simulink model "BMS_Dashboard"  (R2025b)
settings: Solver=FixedStepDiscrete  StartTime=0.0  StopTime=300  FixedStep=Ts  RelTol=1e-3
InitFcn:
  | init_BMS
undefined symbols (not defined in the file): Ts
libraries: BMS_Library x1
settings Model: Creator=Khadija  LastModifiedBy=Khadija

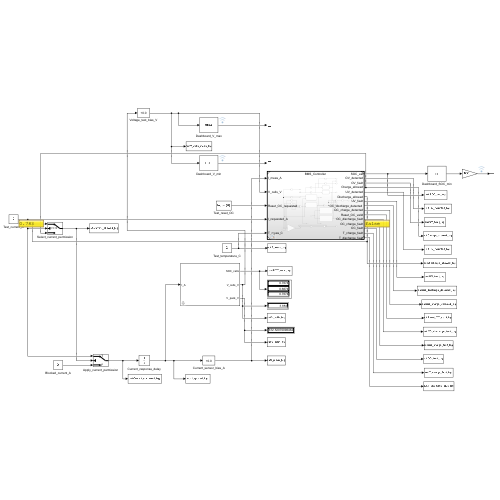
[thumbnail: Simulink's stored preview of the top-level diagram]
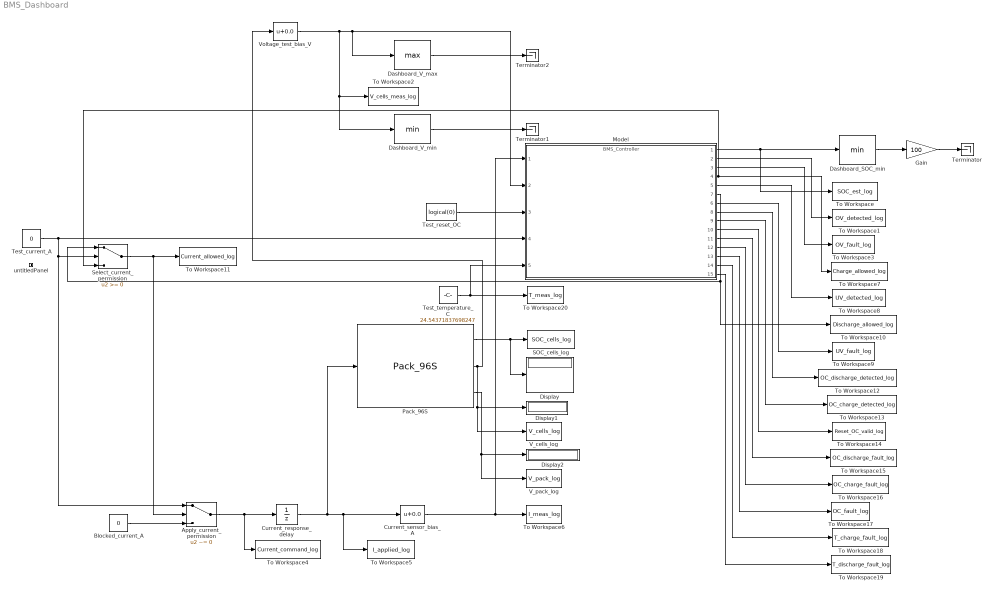
== system BMS_Dashboard ==
  Apply_current_permission : Switch  Criteria=u2 ~= 0  SaturateOnIntegerOverflow=off  InputSameDT=off
  Blocked_current_A : Constant  Value=0  SampleTime=Ts
  Current_response_delay : UnitDelay  SampleTime=Ts  HasFrameUpgradeWarning=on
  Current_sensor_bias_A : Bias  Bias=0.0  SaturateOnIntegerOverflow=off
  Dashboard_SOC_min : MinMax
  Dashboard_V_max : MinMax  Function=max
  Dashboard_V_min : MinMax
  Display : Display
  Display1 : Display
  Display2 : Display
  Gain : Gain  Gain=100
  Model : ModelReference  ModelNameDialog=BMS_Controller  SimulationMode=Normal  ModelReferenceVersion=1.40
      settings: PortSchema="{\"entries\":[{\"content\":{\"sides\":[{\"content\":{\"connectorIds\":[\"In1\",\"In2\",\"In3\",\"In4\",\"In5\"]},\"type\":\"ConnectorPlacement.EquallySpacedRectSide\",\"uuid\":\"1e26f145-0f3d-496d-921d-7ad329268fcb\"},{\"content\":{\"connectorIds\":[\"Out1\",\"Out2\",\"Out3\",\"Out4\",\"Out5\",\"Out7\",\"Out6\",\"Out8\",\"Out9\",\"Out10\",\"Out11\",\"Out12\",\"Out13\",\"Out14\",\"Out15\"],\"side\":\"RIGHT\"},\"type\":\"ConnectorPlacement.EquallySpacedRectSide\",\"uuid\":\"f623cd1b-04b5-4ae4-86fc-b9e653a015f6\"},{\"content\":{\"side\":\"TOP\"},\"type\":\"ConnectorPlacement.EquallySpacedRectSide\",\"uuid\":\"e3a00977-f6c2-4554-bcd2-84dd8f01a2c6\"}]},\"type\":\"ConnectorPlacement.EquallySpacedConnector\",\"uuid\":\"60ffb283-705f-43a9-b3aa-b4ebe7e6c32d\"}],\"packageUris\":[\"http://schema.mathworks.com/mf0/Connector/R2020b\"],\"version\":\"1.0\"}"
  Pack_96S : BMS_Library/Pack_96S  SOC_init_pack=SOC0_pack
  SOC_cells_log : ToWorkspace  VariableName=SOC_cells_log  SaveFormat=Timeseries  SampleTime=-1
  Select_current_permission : Switch  SaturateOnIntegerOverflow=off  InputSameDT=off
  Terminator : Terminator
  Terminator1 : Terminator
  Terminator2 : Terminator
  Test_current_A : Constant  Value=0  SampleTime=Ts
  Test_reset_OC : Constant  Value=logical(0)  SampleTime=Ts
  Test_temperature_C : Constant  Value=24.54371837698247  OutDataTypeStr=double  SampleTime=Ts
  To Workspace : ToWorkspace  VariableName=SOC_est_log  SaveFormat=Timeseries  SampleTime=-1
  To Workspace1 : ToWorkspace  VariableName=OV_detected_log  SaveFormat=Timeseries  SampleTime=-1
  To Workspace10 : ToWorkspace  VariableName=Discharge_allowed_log  SaveFormat=Timeseries  SampleTime=-1
  To Workspace11 : ToWorkspace  VariableName=Current_allowed_log  SaveFormat=Timeseries  SampleTime=-1
  To Workspace12 : ToWorkspace  VariableName=OC_discharge_detected_log  SaveFormat=Timeseries  SampleTime=-1
  To Workspace13 : ToWorkspace  VariableName=OC_charge_detected_log  SaveFormat=Timeseries  SampleTime=-1
  To Workspace14 : ToWorkspace  VariableName=Reset_OC_valid_log  SaveFormat=Timeseries  SampleTime=-1
  To Workspace15 : ToWorkspace  VariableName=OC_discharge_fault_log  SaveFormat=Timeseries  SampleTime=-1
  To Workspace16 : ToWorkspace  VariableName=OC_charge_fault_log  SaveFormat=Timeseries  SampleTime=-1
  To Workspace17 : ToWorkspace  VariableName=OC_fault_log  SaveFormat=Timeseries  SampleTime=-1
  To Workspace18 : ToWorkspace  VariableName=T_charge_fault_log  SaveFormat=Timeseries  SampleTime=-1
  To Workspace19 : ToWorkspace  VariableName=T_discharge_fault_log  SaveFormat=Timeseries  SampleTime=-1
  To Workspace2 : ToWorkspace  VariableName=V_cells_meas_log  SaveFormat=Timeseries  SampleTime=-1
  To Workspace20 : ToWorkspace  VariableName=T_meas_log  SaveFormat=Timeseries  SampleTime=-1
  To Workspace3 : ToWorkspace  VariableName=OV_fault_log  SaveFormat=Timeseries  SampleTime=-1
  To Workspace4 : ToWorkspace  VariableName=Current_command_log  SaveFormat=Timeseries  SampleTime=-1
  To Workspace5 : ToWorkspace  VariableName=I_applied_log  SaveFormat=Timeseries  SampleTime=-1
  To Workspace6 : ToWorkspace  VariableName=I_meas_log  SaveFormat=Timeseries  SampleTime=-1
  To Workspace7 : ToWorkspace  VariableName=Charge_allowed_log  SaveFormat=Timeseries  SampleTime=-1
  To Workspace8 : ToWorkspace  VariableName=UV_detected_log  SaveFormat=Timeseries  SampleTime=-1
  To Workspace9 : ToWorkspace  VariableName=UV_fault_log  SaveFormat=Timeseries  SampleTime=-1
  V_cells_log : ToWorkspace  VariableName=V_cells_log  SaveFormat=Timeseries  SampleTime=-1
  V_pack_log : ToWorkspace  VariableName=V_pack_log  SaveFormat=Timeseries  SampleTime=-1
  Voltage_test_bias_V : Bias  Bias=0.0  SaturateOnIntegerOverflow=off
  untitledPanel : Subsystem  Tag=HiddenForWebPanel  IsWebBlockPanel=on
  wires:
  Test_temperature_C/1 -> Model/5, To Workspace20/1
  Test_current_A/1 -> Apply_current_permission/1, Select_current_permission/2, Model/4
  Select_current_permission/1 -> Apply_current_permission/2, To Workspace11/1
  Apply_current_permission/1 -> Current_response_delay/1, To Workspace4/1
  Blocked_current_A/1 -> Apply_current_permission/3
  Current_response_delay/1 -> To Workspace5/1, Current_sensor_bias_A/1, Pack_96S/1
  Dashboard_V_min/1 -> Terminator1/1
  Dashboard_V_max/1 -> Terminator2/1
  Voltage_test_bias_V/1 -> Dashboard_V_min/1, To Workspace2/1, Model/2, Dashboard_V_max/1
  Test_reset_OC/1 -> Model/3
  Pack_96S/1 -> Display/1, SOC_cells_log/1
  Pack_96S/2 -> V_cells_log/1, Display1/1, Voltage_test_bias_V/1
  Model/15 -> To Workspace19/1
  Pack_96S/3 -> Display2/1, V_pack_log/1
  Current_sensor_bias_A/1 -> Model/1, To Workspace6/1
  Model/13 -> To Workspace17/1
  Model/9 -> To Workspace13/1
  Model/5 -> To Workspace8/1
  Model/1 -> Dashboard_SOC_min/1, To Workspace/1
  Model/14 -> To Workspace18/1
  Model/10 -> To Workspace14/1
  Model/6 -> To Workspace9/1
  Model/2 -> To Workspace1/1
  Model/11 -> To Workspace15/1
  Model/7 -> Select_current_permission/1, To Workspace10/1
  Model/3 -> To Workspace3/1
  Model/12 -> To Workspace16/1
  Model/8 -> To Workspace12/1
  Model/4 -> Select_current_permission/3, To Workspace7/1
  Dashboard_SOC_min/1 -> Gain/1
  Gain/1 -> Terminator/1

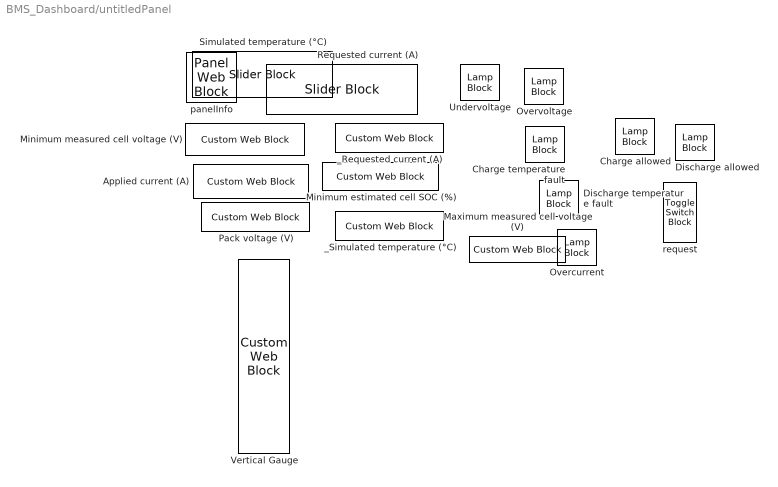
== system BMS_Dashboard/untitledPanel ==
  Applied current (A) : CustomWebBlock  Tag=HiddenForWebPanel  PanelInfo="{\"height\":38,\"left\":371,\"panelId\":\"panelId-01a7e0ec-c42e-414d-a098-7f8dff93f820\",\"top\":179,\"type\":\"panelChild\",\"version\":\"2019b\",\"width\":128,\"zIndex\":1500028}"  LabelPosition=Hide  ShowInitialText=on  Configuration="{\"components\":[{\"name\":\"DisplayComponent\",\"settings\":{\"bold\":false,\"font\":\"DSEG7 Classic\",\"fontColor\":[255,255,200],\"fontSize\":\"7.015042251148508\",\"format\":\"short\",\"formatString\":\"%d\",\"italic\":false,\"position\":[0,0,1,1],\"underline\":false}},{\"name\":\"BackgroundImageComponent\",\"settings\":{\"image\":{\"size\":[300,80],\"src\":\"data:image\\/svg+xml;base64,PHN2ZyBpZD0iZnJhbWUiIHhtbG5zPSJodHRwOi8vd3d3LnczLm9yZy8yMDAwL3N2ZyIgeG1sbnM6eGxpbms9Imh0dHA6Ly93d3cudzMub3JnLzE5OTkveGxpbmsiIHZpZXdCb3g9IjAgMCAzODAgMTAxIj48ZGVmcz48c3R5bGU+LmNscy0xe2ZpbGw6IzAwMmI0Mjt9LmNscy0ye2ZpbGw6IzQyNzA4Mjt9LmNscy0ze2ZpbGw6dXJsKCNyYWRpYWwtZ3JhZGllbnQpO308L3N0eWxlPjxyYWRpYWxHcmFkaWVudCBpZD0icmFkaWFsLWdyYWRpZW50IiBjeD0iMTkwIiBjeT0iNTAuNSIgcj0iMjY5LjIxIiBncmFkaWVudFVuaXRzPSJ1c2VyU3BhY2VPblVzZSI+PHN0b3Agb2Zmc2V0PSIwLjAxIiBzdG9wLWNvbG9yPSIjM2U0ZjU4Ii8+PHN0b3Agb2Zmc2V0PSIwLjA2IiBzdG9wLWNvbG9yPSIjNDQ1NzYxIi8+PHN0b3Agb2Zmc2V0PSIwLjE1IiBzdG9wLWNvbG9yPSIjNTU2YTc2Ii8+PHN0b3Agb2Zmc2V0PSIwLjI1IiBzdG9wLWNvbG9yPSIjNmQ4ODk1Ii8+PHN0b3Agb2Zmc2V0PSIwLjM4IiBzdG9wLWNvbG9yPSIjOGZiMmMzIi8+PHN0b3Agb2Zmc2V0PSIwLjUyIiBzdG9wLWNvbG9yPSIjYjZlNGZhIi8+PHN0b3Agb2Zmc2V0PSIxIiBzdG9wLWNvbG9yPSIjMTU0NjU3Ii8+PC9yYWRpYWxHcmFkaWVudD48L2RlZnM+PGcgaWQ9IkxheWVyXzIiIGRhdGEtbmFtZT0iTGF5ZXIgMiI+PGcgaWQ9IkxheWVyXzEtMiIgZGF0YS1uYW1lPSJMYXllciAxLTIiPjxyZWN0IGlkPSJyZWN0MTAzNiIgY2xhc3M9ImNscy0xIiB4PSIxMSIgeT0iMTEiIHdpZHRoPSIzNTgiIGhlaWdodD0iNzkiLz48cGF0aCBpZD0icGF0aDEwMzgiIGNsYXNzPSJjbHMtMiIgZD0iTTgsOFY5M0gzNzJWOFpNMzY5LDkwSDExVjExSDM2OVoiLz48cGF0aCBpZD0icGF0aDEwNDAiIGNsYXNzPSJjbHMtMyIgZD0iTTAsMFYxMDFIMzgwVjBaTTM3Miw5M0g4VjhIMzcyWiIvPjwvZz48L2c+PC9zdmc+\",\"srcOrientation\":\"Right\"},\"position\":[0,0,1,1],\"scaleMode\":\"0\"}},{\"name\":\"ForegroundImageComponent\",\"settings\":{\"angle\":0,\"image\":{\"size\":[0,0],\"src\":\"default\"},\"isForeground\":1,\"position\":[0,0,1,1],\"scaleMode\":\"0\"}}],\"derived\":{\"blockParameters\":{\"fixedAspectRatio\":\"on\",\"format\":\"short\",\"formatString\":\"%d\"}},\"settings\":{\"BindingType\":\"signal\",\"aspectRatio\":1.032258064516129,\"backgroundColor\":[0,0,0,\"1\"],\"backgroundOffset\":0.14,\"backgroundOpacity\":1,\"fixedAspectRatio\":\"on\",\"showBackgroundColor\":false,\"value\":0,\"version\":\"R2023b\"},\"type\":\"Display\"}"
  Charge allowed : LampBlock  Tag=HiddenForWebPanel  PanelInfo="{\"height\":38,\"left\":335,\"panelId\":\"panelId-01a7e0ec-c42e-414d-a098-7f8dff93f820\",\"top\":304,\"type\":\"panelChild\",\"version\":\"2019b\",\"width\":42,\"zIndex\":1500014}"  DefaultColor=[100.0, 212.0, 19.0]
  Charge temperature fault : LampBlock  Tag=HiddenForWebPanel  PanelInfo="{\"height\":38,\"left\":201,\"panelId\":\"panelId-01a7e0ec-c42e-414d-a098-7f8dff93f820\",\"top\":406,\"type\":\"panelChild\",\"version\":\"2019b\",\"width\":42,\"zIndex\":1500008}"  DefaultColor=[254.0, 51.0, 10.0]
  Discharge allowed : LampBlock  Tag=HiddenForWebPanel  PanelInfo="{\"height\":38,\"left\":460,\"panelId\":\"panelId-01a7e0ec-c42e-414d-a098-7f8dff93f820\",\"top\":303,\"type\":\"panelChild\",\"version\":\"2019b\",\"width\":42,\"zIndex\":1500016}"  DefaultColor=[100.0, 212.0, 19.0]
  Discharge temperature fault : LampBlock  Tag=HiddenForWebPanel  PanelInfo="{\"height\":38,\"left\":511,\"panelId\":\"panelId-01a7e0ec-c42e-414d-a098-7f8dff93f820\",\"top\":405,\"type\":\"panelChild\",\"version\":\"2019b\",\"width\":42,\"zIndex\":1500020}"  DefaultColor=[254.0, 51.0, 10.0]
  Maximum measured cell voltage (V) : CustomWebBlock  Tag=HiddenForWebPanel  PanelInfo="{\"height\":35,\"left\":468,\"panelId\":\"panelId-01a7e0ec-c42e-414d-a098-7f8dff93f820\",\"top\":242,\"type\":\"panelChild\",\"version\":\"2019b\",\"width\":128,\"zIndex\":1500034}"  LabelPosition=Hide  ShowInitialText=on  Configuration="{\"components\":[{\"name\":\"DisplayComponent\",\"settings\":{\"bold\":false,\"font\":\"DSEG7 Classic\",\"fontColor\":[255,255,200],\"fontSize\":\"7.015042251148508\",\"format\":\"short\",\"formatString\":\"%d\",\"italic\":false,\"position\":[0,0,1,1],\"underline\":false}},{\"name\":\"BackgroundImageComponent\",\"settings\":{\"image\":{\"size\":[300,80],\"src\":\"data:image\\/svg+xml;base64,PHN2ZyBpZD0iZnJhbWUiIHhtbG5zPSJodHRwOi8vd3d3LnczLm9yZy8yMDAwL3N2ZyIgeG1sbnM6eGxpbms9Imh0dHA6Ly93d3cudzMub3JnLzE5OTkveGxpbmsiIHZpZXdCb3g9IjAgMCAzODAgMTAxIj48ZGVmcz48c3R5bGU+LmNscy0xe2ZpbGw6IzAwMmI0Mjt9LmNscy0ye2ZpbGw6IzQyNzA4Mjt9LmNscy0ze2ZpbGw6dXJsKCNyYWRpYWwtZ3JhZGllbnQpO308L3N0eWxlPjxyYWRpYWxHcmFkaWVudCBpZD0icmFkaWFsLWdyYWRpZW50IiBjeD0iMTkwIiBjeT0iNTAuNSIgcj0iMjY5LjIxIiBncmFkaWVudFVuaXRzPSJ1c2VyU3BhY2VPblVzZSI+PHN0b3Agb2Zmc2V0PSIwLjAxIiBzdG9wLWNvbG9yPSIjM2U0ZjU4Ii8+PHN0b3Agb2Zmc2V0PSIwLjA2IiBzdG9wLWNvbG9yPSIjNDQ1NzYxIi8+PHN0b3Agb2Zmc2V0PSIwLjE1IiBzdG9wLWNvbG9yPSIjNTU2YTc2Ii8+PHN0b3Agb2Zmc2V0PSIwLjI1IiBzdG9wLWNvbG9yPSIjNmQ4ODk1Ii8+PHN0b3Agb2Zmc2V0PSIwLjM4IiBzdG9wLWNvbG9yPSIjOGZiMmMzIi8+PHN0b3Agb2Zmc2V0PSIwLjUyIiBzdG9wLWNvbG9yPSIjYjZlNGZhIi8+PHN0b3Agb2Zmc2V0PSIxIiBzdG9wLWNvbG9yPSIjMTU0NjU3Ii8+PC9yYWRpYWxHcmFkaWVudD48L2RlZnM+PGcgaWQ9IkxheWVyXzIiIGRhdGEtbmFtZT0iTGF5ZXIgMiI+PGcgaWQ9IkxheWVyXzEtMiIgZGF0YS1uYW1lPSJMYXllciAxLTIiPjxyZWN0IGlkPSJyZWN0MTAzNiIgY2xhc3M9ImNscy0xIiB4PSIxMSIgeT0iMTEiIHdpZHRoPSIzNTgiIGhlaWdodD0iNzkiLz48cGF0aCBpZD0icGF0aDEwMzgiIGNsYXNzPSJjbHMtMiIgZD0iTTgsOFY5M0gzNzJWOFpNMzY5LDkwSDExVjExSDM2OVoiLz48cGF0aCBpZD0icGF0aDEwNDAiIGNsYXNzPSJjbHMtMyIgZD0iTTAsMFYxMDFIMzgwVjBaTTM3Miw5M0g4VjhIMzcyWiIvPjwvZz48L2c+PC9zdmc+\",\"srcOrientation\":\"Right\"},\"position\":[0,0,1,1],\"scaleMode\":\"0\"}},{\"name\":\"ForegroundImageComponent\",\"settings\":{\"angle\":0,\"image\":{\"size\":[0,0],\"src\":\"default\"},\"isForeground\":1,\"position\":[0,0,1,1],\"scaleMode\":\"0\"}}],\"derived\":{\"blockParameters\":{\"fixedAspectRatio\":\"on\",\"format\":\"short\",\"formatString\":\"%d\"}},\"settings\":{\"BindingType\":\"signal\",\"aspectRatio\":1.032258064516129,\"backgroundColor\":[0,0,0,\"1\"],\"backgroundOffset\":0.14,\"backgroundOpacity\":1,\"fixedAspectRatio\":\"on\",\"showBackgroundColor\":false,\"value\":0,\"version\":\"R2023b\"},\"type\":\"Display\"}"
  Minimum estimated cell SOC (%) : CustomWebBlock  Tag=HiddenForWebPanel  PanelInfo="{\"height\":35,\"left\":36,\"panelId\":\"panelId-01a7e0ec-c42e-414d-a098-7f8dff93f820\",\"top\":182,\"type\":\"panelChild\",\"version\":\"2019b\",\"width\":145,\"zIndex\":1500026}"  LabelPosition=Hide  ShowInitialText=on  Configuration="{\"components\":[{\"name\":\"DisplayComponent\",\"settings\":{\"bold\":false,\"font\":\"DSEG7 Classic\",\"fontColor\":[255,255,200],\"fontSize\":\"7.015042251148508\",\"format\":\"short\",\"formatString\":\"%d\",\"italic\":false,\"position\":[0,0,1,1],\"underline\":false}},{\"name\":\"BackgroundImageComponent\",\"settings\":{\"image\":{\"size\":[300,80],\"src\":\"data:image\\/svg+xml;base64,PHN2ZyBpZD0iZnJhbWUiIHhtbG5zPSJodHRwOi8vd3d3LnczLm9yZy8yMDAwL3N2ZyIgeG1sbnM6eGxpbms9Imh0dHA6Ly93d3cudzMub3JnLzE5OTkveGxpbmsiIHZpZXdCb3g9IjAgMCAzODAgMTAxIj48ZGVmcz48c3R5bGU+LmNscy0xe2ZpbGw6IzAwMmI0Mjt9LmNscy0ye2ZpbGw6IzQyNzA4Mjt9LmNscy0ze2ZpbGw6dXJsKCNyYWRpYWwtZ3JhZGllbnQpO308L3N0eWxlPjxyYWRpYWxHcmFkaWVudCBpZD0icmFkaWFsLWdyYWRpZW50IiBjeD0iMTkwIiBjeT0iNTAuNSIgcj0iMjY5LjIxIiBncmFkaWVudFVuaXRzPSJ1c2VyU3BhY2VPblVzZSI+PHN0b3Agb2Zmc2V0PSIwLjAxIiBzdG9wLWNvbG9yPSIjM2U0ZjU4Ii8+PHN0b3Agb2Zmc2V0PSIwLjA2IiBzdG9wLWNvbG9yPSIjNDQ1NzYxIi8+PHN0b3Agb2Zmc2V0PSIwLjE1IiBzdG9wLWNvbG9yPSIjNTU2YTc2Ii8+PHN0b3Agb2Zmc2V0PSIwLjI1IiBzdG9wLWNvbG9yPSIjNmQ4ODk1Ii8+PHN0b3Agb2Zmc2V0PSIwLjM4IiBzdG9wLWNvbG9yPSIjOGZiMmMzIi8+PHN0b3Agb2Zmc2V0PSIwLjUyIiBzdG9wLWNvbG9yPSIjYjZlNGZhIi8+PHN0b3Agb2Zmc2V0PSIxIiBzdG9wLWNvbG9yPSIjMTU0NjU3Ii8+PC9yYWRpYWxHcmFkaWVudD48L2RlZnM+PGcgaWQ9IkxheWVyXzIiIGRhdGEtbmFtZT0iTGF5ZXIgMiI+PGcgaWQ9IkxheWVyXzEtMiIgZGF0YS1uYW1lPSJMYXllciAxLTIiPjxyZWN0IGlkPSJyZWN0MTAzNiIgY2xhc3M9ImNscy0xIiB4PSIxMSIgeT0iMTEiIHdpZHRoPSIzNTgiIGhlaWdodD0iNzkiLz48cGF0aCBpZD0icGF0aDEwMzgiIGNsYXNzPSJjbHMtMiIgZD0iTTgsOFY5M0gzNzJWOFpNMzY5LDkwSDExVjExSDM2OVoiLz48cGF0aCBpZD0icGF0aDEwNDAiIGNsYXNzPSJjbHMtMyIgZD0iTTAsMFYxMDFIMzgwVjBaTTM3Miw5M0g4VjhIMzcyWiIvPjwvZz48L2c+PC9zdmc+\",\"srcOrientation\":\"Right\"},\"position\":[0,0,1,1],\"scaleMode\":\"0\"}},{\"name\":\"ForegroundImageComponent\",\"settings\":{\"angle\":0,\"image\":{\"size\":[0,0],\"src\":\"default\"},\"isForeground\":1,\"position\":[0,0,1,1],\"scaleMode\":\"0\"}}],\"derived\":{\"blockParameters\":{\"fixedAspectRatio\":\"on\",\"format\":\"short\",\"formatString\":\"%d\"}},\"settings\":{\"BindingType\":\"signal\",\"aspectRatio\":1.032258064516129,\"backgroundColor\":[0,0,0,\"1\"],\"backgroundOffset\":0.14,\"backgroundOpacity\":1,\"fixedAspectRatio\":\"on\",\"showBackgroundColor\":false,\"value\":0,\"version\":\"R2023b\"},\"type\":\"Display\"}"
  Minimum measured cell voltage (V) : CustomWebBlock  Tag=HiddenForWebPanel  PanelInfo="{\"height\":37,\"left\":528,\"panelId\":\"panelId-01a7e0ec-c42e-414d-a098-7f8dff93f820\",\"top\":179,\"type\":\"panelChild\",\"version\":\"2019b\",\"width\":141,\"zIndex\":1500024}"  LabelPosition=Hide  ShowInitialText=on  Configuration="{\"components\":[{\"name\":\"DisplayComponent\",\"settings\":{\"bold\":false,\"font\":\"DSEG7 Classic\",\"fontColor\":[255,255,200],\"fontSize\":\"7.015042251148508\",\"format\":\"short\",\"formatString\":\"%d\",\"italic\":false,\"position\":[0,0,1,1],\"underline\":false}},{\"name\":\"BackgroundImageComponent\",\"settings\":{\"image\":{\"size\":[300,80],\"src\":\"data:image\\/svg+xml;base64,PHN2ZyBpZD0iZnJhbWUiIHhtbG5zPSJodHRwOi8vd3d3LnczLm9yZy8yMDAwL3N2ZyIgeG1sbnM6eGxpbms9Imh0dHA6Ly93d3cudzMub3JnLzE5OTkveGxpbmsiIHZpZXdCb3g9IjAgMCAzODAgMTAxIj48ZGVmcz48c3R5bGU+LmNscy0xe2ZpbGw6IzAwMmI0Mjt9LmNscy0ye2ZpbGw6IzQyNzA4Mjt9LmNscy0ze2ZpbGw6dXJsKCNyYWRpYWwtZ3JhZGllbnQpO308L3N0eWxlPjxyYWRpYWxHcmFkaWVudCBpZD0icmFkaWFsLWdyYWRpZW50IiBjeD0iMTkwIiBjeT0iNTAuNSIgcj0iMjY5LjIxIiBncmFkaWVudFVuaXRzPSJ1c2VyU3BhY2VPblVzZSI+PHN0b3Agb2Zmc2V0PSIwLjAxIiBzdG9wLWNvbG9yPSIjM2U0ZjU4Ii8+PHN0b3Agb2Zmc2V0PSIwLjA2IiBzdG9wLWNvbG9yPSIjNDQ1NzYxIi8+PHN0b3Agb2Zmc2V0PSIwLjE1IiBzdG9wLWNvbG9yPSIjNTU2YTc2Ii8+PHN0b3Agb2Zmc2V0PSIwLjI1IiBzdG9wLWNvbG9yPSIjNmQ4ODk1Ii8+PHN0b3Agb2Zmc2V0PSIwLjM4IiBzdG9wLWNvbG9yPSIjOGZiMmMzIi8+PHN0b3Agb2Zmc2V0PSIwLjUyIiBzdG9wLWNvbG9yPSIjYjZlNGZhIi8+PHN0b3Agb2Zmc2V0PSIxIiBzdG9wLWNvbG9yPSIjMTU0NjU3Ii8+PC9yYWRpYWxHcmFkaWVudD48L2RlZnM+PGcgaWQ9IkxheWVyXzIiIGRhdGEtbmFtZT0iTGF5ZXIgMiI+PGcgaWQ9IkxheWVyXzEtMiIgZGF0YS1uYW1lPSJMYXllciAxLTIiPjxyZWN0IGlkPSJyZWN0MTAzNiIgY2xhc3M9ImNscy0xIiB4PSIxMSIgeT0iMTEiIHdpZHRoPSIzNTgiIGhlaWdodD0iNzkiLz48cGF0aCBpZD0icGF0aDEwMzgiIGNsYXNzPSJjbHMtMiIgZD0iTTgsOFY5M0gzNzJWOFpNMzY5LDkwSDExVjExSDM2OVoiLz48cGF0aCBpZD0icGF0aDEwNDAiIGNsYXNzPSJjbHMtMyIgZD0iTTAsMFYxMDFIMzgwVjBaTTM3Miw5M0g4VjhIMzcyWiIvPjwvZz48L2c+PC9zdmc+\",\"srcOrientation\":\"Right\"},\"position\":[0,0,1,1],\"scaleMode\":\"0\"}},{\"name\":\"ForegroundImageComponent\",\"settings\":{\"angle\":0,\"image\":{\"size\":[0,0],\"src\":\"default\"},\"isForeground\":1,\"position\":[0,0,1,1],\"scaleMode\":\"0\"}}],\"derived\":{\"blockParameters\":{\"fixedAspectRatio\":\"on\",\"format\":\"short\",\"formatString\":\"%d\"}},\"settings\":{\"BindingType\":\"signal\",\"aspectRatio\":1.032258064516129,\"backgroundColor\":[0,0,0,\"1\"],\"backgroundOffset\":0.14,\"backgroundOpacity\":1,\"fixedAspectRatio\":\"on\",\"showBackgroundColor\":false,\"value\":0,\"version\":\"R2023b\"},\"type\":\"Display\"}"
  Overcurrent : LampBlock  Tag=HiddenForWebPanel  PanelInfo="{\"height\":38,\"left\":779,\"panelId\":\"panelId-01a7e0ec-c42e-414d-a098-7f8dff93f820\",\"top\":406,\"type\":\"panelChild\",\"version\":\"2019b\",\"width\":42,\"zIndex\":1500036}"  DefaultColor=[254.0, 51.0, 10.0]
  Overvoltage : LampBlock  Tag=HiddenForWebPanel  PanelInfo="{\"height\":38,\"left\":372,\"panelId\":\"panelId-01a7e0ec-c42e-414d-a098-7f8dff93f820\",\"top\":405,\"type\":\"panelChild\",\"version\":\"2019b\",\"width\":42,\"zIndex\":1500004}"  DefaultColor=[254.0, 51.0, 10.0]
  Pack voltage (V) : CustomWebBlock  Tag=HiddenForWebPanel  PanelInfo="{\"height\":37,\"left\":688,\"panelId\":\"panelId-01a7e0ec-c42e-414d-a098-7f8dff93f820\",\"top\":178,\"type\":\"panelChild\",\"version\":\"2019b\",\"width\":141,\"zIndex\":1500032}"  LabelPosition=Hide  ShowInitialText=on  Configuration="{\"components\":[{\"name\":\"DisplayComponent\",\"settings\":{\"bold\":false,\"font\":\"DSEG7 Classic\",\"fontColor\":[255,255,200],\"fontSize\":\"7.015042251148508\",\"format\":\"short\",\"formatString\":\"%d\",\"italic\":false,\"position\":[0,0,1,1],\"underline\":false}},{\"name\":\"BackgroundImageComponent\",\"settings\":{\"image\":{\"size\":[300,80],\"src\":\"data:image\\/svg+xml;base64,PHN2ZyBpZD0iZnJhbWUiIHhtbG5zPSJodHRwOi8vd3d3LnczLm9yZy8yMDAwL3N2ZyIgeG1sbnM6eGxpbms9Imh0dHA6Ly93d3cudzMub3JnLzE5OTkveGxpbmsiIHZpZXdCb3g9IjAgMCAzODAgMTAxIj48ZGVmcz48c3R5bGU+LmNscy0xe2ZpbGw6IzAwMmI0Mjt9LmNscy0ye2ZpbGw6IzQyNzA4Mjt9LmNscy0ze2ZpbGw6dXJsKCNyYWRpYWwtZ3JhZGllbnQpO308L3N0eWxlPjxyYWRpYWxHcmFkaWVudCBpZD0icmFkaWFsLWdyYWRpZW50IiBjeD0iMTkwIiBjeT0iNTAuNSIgcj0iMjY5LjIxIiBncmFkaWVudFVuaXRzPSJ1c2VyU3BhY2VPblVzZSI+PHN0b3Agb2Zmc2V0PSIwLjAxIiBzdG9wLWNvbG9yPSIjM2U0ZjU4Ii8+PHN0b3Agb2Zmc2V0PSIwLjA2IiBzdG9wLWNvbG9yPSIjNDQ1NzYxIi8+PHN0b3Agb2Zmc2V0PSIwLjE1IiBzdG9wLWNvbG9yPSIjNTU2YTc2Ii8+PHN0b3Agb2Zmc2V0PSIwLjI1IiBzdG9wLWNvbG9yPSIjNmQ4ODk1Ii8+PHN0b3Agb2Zmc2V0PSIwLjM4IiBzdG9wLWNvbG9yPSIjOGZiMmMzIi8+PHN0b3Agb2Zmc2V0PSIwLjUyIiBzdG9wLWNvbG9yPSIjYjZlNGZhIi8+PHN0b3Agb2Zmc2V0PSIxIiBzdG9wLWNvbG9yPSIjMTU0NjU3Ii8+PC9yYWRpYWxHcmFkaWVudD48L2RlZnM+PGcgaWQ9IkxheWVyXzIiIGRhdGEtbmFtZT0iTGF5ZXIgMiI+PGcgaWQ9IkxheWVyXzEtMiIgZGF0YS1uYW1lPSJMYXllciAxLTIiPjxyZWN0IGlkPSJyZWN0MTAzNiIgY2xhc3M9ImNscy0xIiB4PSIxMSIgeT0iMTEiIHdpZHRoPSIzNTgiIGhlaWdodD0iNzkiLz48cGF0aCBpZD0icGF0aDEwMzgiIGNsYXNzPSJjbHMtMiIgZD0iTTgsOFY5M0gzNzJWOFpNMzY5LDkwSDExVjExSDM2OVoiLz48cGF0aCBpZD0icGF0aDEwNDAiIGNsYXNzPSJjbHMtMyIgZD0iTTAsMFYxMDFIMzgwVjBaTTM3Miw5M0g4VjhIMzcyWiIvPjwvZz48L2c+PC9zdmc+\",\"srcOrientation\":\"Right\"},\"position\":[0,0,1,1],\"scaleMode\":\"0\"}},{\"name\":\"ForegroundImageComponent\",\"settings\":{\"angle\":0,\"image\":{\"size\":[0,0],\"src\":\"default\"},\"isForeground\":1,\"position\":[0,0,1,1],\"scaleMode\":\"0\"}}],\"derived\":{\"blockParameters\":{\"fixedAspectRatio\":\"on\",\"format\":\"short\",\"formatString\":\"%d\"}},\"settings\":{\"BindingType\":\"signal\",\"aspectRatio\":1.032258064516129,\"backgroundColor\":[0,0,0,\"1\"],\"backgroundOffset\":0.14,\"backgroundOpacity\":1,\"fixedAspectRatio\":\"on\",\"showBackgroundColor\":false,\"value\":0,\"version\":\"R2023b\"},\"type\":\"Display\"}"
  Requested current (A) : SliderBlock  Tag=HiddenForWebPanel  PanelInfo="{\"height\":88,\"left\":307,\"panelId\":\"panelId-01a7e0ec-c42e-414d-a098-7f8dff93f820\",\"top\":53,\"type\":\"panelChild\",\"version\":\"2019b\",\"width\":232,\"zIndex\":1500012}"  ScaleMin=-1.5  ScaleMax=2.5  TickInterval=0.5
  Simulated temperature (°C) : SliderBlock  Tag=HiddenForWebPanel  PanelInfo="{\"height\":92,\"left\":65,\"panelId\":\"panelId-01a7e0ec-c42e-414d-a098-7f8dff93f820\",\"top\":52,\"type\":\"panelChild\",\"version\":\"2019b\",\"width\":234,\"zIndex\":1500002}"  ScaleMin=-25  ScaleMax=65
  Undervoltage : LampBlock  Tag=HiddenForWebPanel  PanelInfo="{\"height\":38,\"left\":661,\"panelId\":\"panelId-01a7e0ec-c42e-414d-a098-7f8dff93f820\",\"top\":407,\"type\":\"panelChild\",\"version\":\"2019b\",\"width\":42,\"zIndex\":1500006}"  DefaultColor=[254.0, 51.0, 10.0]
  Vertical Gauge : CustomWebBlock  Tag=HiddenForWebPanel  PanelInfo="{\"height\":194,\"left\":78,\"panelId\":\"panelId-01a7e0ec-c42e-414d-a098-7f8dff93f820\",\"top\":233,\"type\":\"panelChild\",\"version\":\"2019b\",\"width\":51,\"zIndex\":1500038}"  LabelPosition=Bottom  ShowInitialText=on  Configuration="{\"components\":[{\"name\":\"LinearScaleComponent\",\"settings\":{\"bounds\":{\"max\":100,\"min\":0,\"tickInterval\":10},\"internalTickHeightScaleFactor\":0.5,\"labelColor\":[255,255,200],\"labelFont\":{\"font\":\"Arial\",\"fontSize\":12},\"labelOffset\":0.05,\"labelTransparency\":1,\"needleImage\":{\"size\":[21,75],\"src\":\"data:image\\/svg+xml;base64,PHN2ZyB4bWxucz0iaHR0cDovL3d3dy53My5vcmcvMjAwMC9zdmciIHhtbG5zOnhsaW5rPSJodHRwOi8vd3d3LnczLm9yZy8xOTk5L3hsaW5rIiB2aWV3Qm94PSIwIDAgMjEgNzUiPjxkZWZzPjxzdHlsZT4uY2xzLTF7ZmlsbDpub25lO30uY2xzLTJ7aXNvbGF0aW9uOmlzb2xhdGU7fS5jbHMtM3tjbGlwLXBhdGg6dXJsKCNjbGlwLXBhdGgpO30uY2xzLTR7b3BhY2l0eTowLjM7bWl4LWJsZW5kLW1vZGU6bXVsdGlwbHk7fS5jbHMtNXtmaWxsOiNlYjI2Mjk7fTwvc3R5bGU+PGNsaXBQYXRoIGlkPSJjbGlwLXBhdGgiIHRyYW5zZm9y ...(+1928 chars)\",\"srcOrientation\":\"horizontal\"},\"needleOffset\":[0.007413509060955519,0],\"needleSize\":{\"height\":0.11955094537815127,\"width\":0.7589285714285714},\"position\":[0.015821953781512604,0.06944444444444445,0.7996031746031746,0.9641544117647058],\"referencePoint\":\"auto\",\"scaleColors\":[],\"scaleColorsSize\":0.2,\"scaleDirection\":\"BT\",\"showLabels\":1,\"showMinorTicks\":0,\"showSpanLine\":1,\"showTicks\":1,\"tickColor\":[252,252,197],\"tickTransparency\":1,\"valueBarColor\":[0,255,0],\"valueBarOffset\":0,\"valueBarSize\":0.7,\"valueBarTransparency\":1}},{\"name\":\"BackgroundImageComponent\",\"settings\":{\"image\":{\"size\":[380,101],\"src\":\"data:image\\/svg+xml;base64,PHN2ZyBpZD0iZnJhbWUiIHhtbG5zPSJodHRwOi8vd3d3LnczLm9yZy8yMDAwL3N2ZyIgeG1sbnM6eGxpbms9Imh0dHA6Ly93d3cudzMub3JnLzE5OTkveGxpbmsiIHZpZXdCb3g9IjAgMCAzODAgMTAxIj48ZGVmcz48c3R5bGU+LmNscy0xe2ZpbGw6IzAwMmI0Mjt9LmNscy0ye2ZpbGw6IzQyNzA4Mjt9LmNscy0ze2ZpbGw6dXJsKCNyYWRpYWwtZ3JhZGllbnQpO308L3N0eWxlPjxyYWRpYWxHcmFkaWVudCBpZD0icmFkaWFsLWdyYWRpZW50IiBjeD0iMTkwIiBjeT0iNTAuNSIgcj0iMjY5LjIxIiBncmFkaWVudFVuaXRzPSJ1c2VyU3BhY2VPblVzZSI+PHN0b3Agb2Zmc2V0PSIwLjAxIiBzdG9wLWNvbG9yPSIjM2U0ZjU4Ii8+PHN0b3Agb2Zmc2V0PSIwLjA2IiBzdG9wLWNvbG9yPSIjNDQ1NzYxIi8+PHN0b3Agb2Zmc2V0PSIwLjE1IiBzdG9wLWNvbG9yPSIjNTU2YTc2Ii8+PHN0b3Agb2Zmc2V0PSIwLjI1IiBzdG9wLWNvbG9yPSIjNmQ4ODk1Ii8+PHN0b3Agb2Zmc2V0PSIwLjM4IiBzdG9wLWNvbG9yPSIjOGZiMmMzIi8+PHN0b3Agb2Zmc2V0PSIwLjUyIiBzdG9wLWNvbG9yPSIjYjZlNGZhIi8+PHN0b3Agb2Zmc2V0PSIxIiBzdG9wLWNvbG9yPSIjMTU0NjU3Ii8+PC9yYWRpYWxHcmFkaWVudD48L2RlZnM+PGcgaWQ9IkxheWVyXzIiIGRhdGEtbmFtZT0iTGF5ZXIgMiI+PGcgaWQ9IkxheWVyXzEtMiIgZGF0YS1uYW1lPSJMYXllciAxLTIiPjxyZWN0IGlkPSJyZWN0MTAzNiIgY2xhc3M9ImNscy0xIiB4PSIxMSIgeT0iMTEiIHdpZHRoPSIzNTgiIGhlaWdodD0iNzkiLz48cGF0aCBpZD0icGF0aDEwMzgiIGNsYXNzPSJjbHMtMiIgZD0iTTgsOFY5M0gzNzJWOFpNMzY5LDkwSDExVjExSDM2OVoiLz48cGF0aCBpZD0icGF0aDEwNDAiIGNsYXNzPSJjbHMtMyIgZD0iTTAsMFYxMDFIMzgwVjBaTTM3Miw5M0g4VjhIMzcyWiIvPjwvZz48L2c+PC9zdmc+\",\"srcOrientation\":\"horizontal\"},\"position\":[0,0,1,1],\"scaleMode\":\"0\"}},{\"name\":\"ForegroundImageComponent\",\"settings\":{\"image\":{\"size\":[0,0],\"src\":\"default\",\"srcOrientation\":[]},\"isForeground\":1,\"position\":[0,0,1,1],\"scaleMode\":\"0\"}}],\"derived\":{\"blockParameters\":{\"ForegroundColor\":[0.9882352941176471,0.9882352941176471,0.7725490196078432],\"Limits\":{\"Max\":100,\"Min\":0,\"Ticks\":10},\"ScaleColors\":[],\"ScaleDirection\":\"Clockwise\",\"ScaleMax\":100,\"ScaleMin\":0,\"TickInterval\":10,\"fixedAspectRatio\":\"on\"}},\"settings\":{\"BindingType\":\"signal\",\"backgroundColor\":[0,0,0,\"1\"],\"backgroundOffset\":0,\"backgroundOpacity\":1,\"fixedAspectRatio\":\"on\",\"orientation\":\"vertical\",\"showBackgroundColor\":false,\"value\":0,\"version\":\"R2023a\"},\"type\":\"LinearGauge\"}"
  _Requested current (A) : CustomWebBlock  Tag=HiddenForWebPanel  PanelInfo="{\"height\":35,\"left\":219,\"panelId\":\"panelId-01a7e0ec-c42e-414d-a098-7f8dff93f820\",\"top\":182,\"type\":\"panelChild\",\"version\":\"2019b\",\"width\":130,\"zIndex\":1500022}"  LabelPosition=Hide  ShowInitialText=on  Configuration="{\"components\":[{\"name\":\"DisplayComponent\",\"settings\":{\"bold\":false,\"font\":\"DSEG7 Classic\",\"fontColor\":[255,255,200],\"fontSize\":\"7.015042251148508\",\"format\":\"short\",\"formatString\":\"%d\",\"italic\":false,\"position\":[0,0,1,1],\"underline\":false}},{\"name\":\"BackgroundImageComponent\",\"settings\":{\"image\":{\"size\":[300,80],\"src\":\"data:image\\/svg+xml;base64,PHN2ZyBpZD0iZnJhbWUiIHhtbG5zPSJodHRwOi8vd3d3LnczLm9yZy8yMDAwL3N2ZyIgeG1sbnM6eGxpbms9Imh0dHA6Ly93d3cudzMub3JnLzE5OTkveGxpbmsiIHZpZXdCb3g9IjAgMCAzODAgMTAxIj48ZGVmcz48c3R5bGU+LmNscy0xe2ZpbGw6IzAwMmI0Mjt9LmNscy0ye2ZpbGw6IzQyNzA4Mjt9LmNscy0ze2ZpbGw6dXJsKCNyYWRpYWwtZ3JhZGllbnQpO308L3N0eWxlPjxyYWRpYWxHcmFkaWVudCBpZD0icmFkaWFsLWdyYWRpZW50IiBjeD0iMTkwIiBjeT0iNTAuNSIgcj0iMjY5LjIxIiBncmFkaWVudFVuaXRzPSJ1c2VyU3BhY2VPblVzZSI+PHN0b3Agb2Zmc2V0PSIwLjAxIiBzdG9wLWNvbG9yPSIjM2U0ZjU4Ii8+PHN0b3Agb2Zmc2V0PSIwLjA2IiBzdG9wLWNvbG9yPSIjNDQ1NzYxIi8+PHN0b3Agb2Zmc2V0PSIwLjE1IiBzdG9wLWNvbG9yPSIjNTU2YTc2Ii8+PHN0b3Agb2Zmc2V0PSIwLjI1IiBzdG9wLWNvbG9yPSIjNmQ4ODk1Ii8+PHN0b3Agb2Zmc2V0PSIwLjM4IiBzdG9wLWNvbG9yPSIjOGZiMmMzIi8+PHN0b3Agb2Zmc2V0PSIwLjUyIiBzdG9wLWNvbG9yPSIjYjZlNGZhIi8+PHN0b3Agb2Zmc2V0PSIxIiBzdG9wLWNvbG9yPSIjMTU0NjU3Ii8+PC9yYWRpYWxHcmFkaWVudD48L2RlZnM+PGcgaWQ9IkxheWVyXzIiIGRhdGEtbmFtZT0iTGF5ZXIgMiI+PGcgaWQ9IkxheWVyXzEtMiIgZGF0YS1uYW1lPSJMYXllciAxLTIiPjxyZWN0IGlkPSJyZWN0MTAzNiIgY2xhc3M9ImNscy0xIiB4PSIxMSIgeT0iMTEiIHdpZHRoPSIzNTgiIGhlaWdodD0iNzkiLz48cGF0aCBpZD0icGF0aDEwMzgiIGNsYXNzPSJjbHMtMiIgZD0iTTgsOFY5M0gzNzJWOFpNMzY5LDkwSDExVjExSDM2OVoiLz48cGF0aCBpZD0icGF0aDEwNDAiIGNsYXNzPSJjbHMtMyIgZD0iTTAsMFYxMDFIMzgwVjBaTTM3Miw5M0g4VjhIMzcyWiIvPjwvZz48L2c+PC9zdmc+\",\"srcOrientation\":\"Right\"},\"position\":[0,0,1,1],\"scaleMode\":\"0\"}},{\"name\":\"ForegroundImageComponent\",\"settings\":{\"angle\":0,\"image\":{\"size\":[0,0],\"src\":\"default\"},\"isForeground\":1,\"position\":[0,0,1,1],\"scaleMode\":\"0\"}}],\"derived\":{\"blockParameters\":{\"fixedAspectRatio\":\"on\",\"format\":\"short\",\"formatString\":\"%d\"}},\"settings\":{\"BindingType\":\"signal\",\"aspectRatio\":1.032258064516129,\"backgroundColor\":[0,0,0,\"1\"],\"backgroundOffset\":0.14,\"backgroundOpacity\":1,\"fixedAspectRatio\":\"on\",\"showBackgroundColor\":false,\"value\":0,\"version\":\"R2023b\"},\"type\":\"Display\"}"
  _Simulated temperature (°C) : CustomWebBlock  Tag=HiddenForWebPanel  PanelInfo="{\"height\":33,\"left\":272,\"panelId\":\"panelId-01a7e0ec-c42e-414d-a098-7f8dff93f820\",\"top\":244,\"type\":\"panelChild\",\"version\":\"2019b\",\"width\":123,\"zIndex\":1500030}"  LabelPosition=Hide  ShowInitialText=on  Configuration="{\"components\":[{\"name\":\"DisplayComponent\",\"settings\":{\"bold\":false,\"font\":\"DSEG7 Classic\",\"fontColor\":[255,255,200],\"fontSize\":\"7.015042251148508\",\"format\":\"short\",\"formatString\":\"%d\",\"italic\":false,\"position\":[0,0,1,1],\"underline\":false}},{\"name\":\"BackgroundImageComponent\",\"settings\":{\"image\":{\"size\":[300,80],\"src\":\"data:image\\/svg+xml;base64,PHN2ZyBpZD0iZnJhbWUiIHhtbG5zPSJodHRwOi8vd3d3LnczLm9yZy8yMDAwL3N2ZyIgeG1sbnM6eGxpbms9Imh0dHA6Ly93d3cudzMub3JnLzE5OTkveGxpbmsiIHZpZXdCb3g9IjAgMCAzODAgMTAxIj48ZGVmcz48c3R5bGU+LmNscy0xe2ZpbGw6IzAwMmI0Mjt9LmNscy0ye2ZpbGw6IzQyNzA4Mjt9LmNscy0ze2ZpbGw6dXJsKCNyYWRpYWwtZ3JhZGllbnQpO308L3N0eWxlPjxyYWRpYWxHcmFkaWVudCBpZD0icmFkaWFsLWdyYWRpZW50IiBjeD0iMTkwIiBjeT0iNTAuNSIgcj0iMjY5LjIxIiBncmFkaWVudFVuaXRzPSJ1c2VyU3BhY2VPblVzZSI+PHN0b3Agb2Zmc2V0PSIwLjAxIiBzdG9wLWNvbG9yPSIjM2U0ZjU4Ii8+PHN0b3Agb2Zmc2V0PSIwLjA2IiBzdG9wLWNvbG9yPSIjNDQ1NzYxIi8+PHN0b3Agb2Zmc2V0PSIwLjE1IiBzdG9wLWNvbG9yPSIjNTU2YTc2Ii8+PHN0b3Agb2Zmc2V0PSIwLjI1IiBzdG9wLWNvbG9yPSIjNmQ4ODk1Ii8+PHN0b3Agb2Zmc2V0PSIwLjM4IiBzdG9wLWNvbG9yPSIjOGZiMmMzIi8+PHN0b3Agb2Zmc2V0PSIwLjUyIiBzdG9wLWNvbG9yPSIjYjZlNGZhIi8+PHN0b3Agb2Zmc2V0PSIxIiBzdG9wLWNvbG9yPSIjMTU0NjU3Ii8+PC9yYWRpYWxHcmFkaWVudD48L2RlZnM+PGcgaWQ9IkxheWVyXzIiIGRhdGEtbmFtZT0iTGF5ZXIgMiI+PGcgaWQ9IkxheWVyXzEtMiIgZGF0YS1uYW1lPSJMYXllciAxLTIiPjxyZWN0IGlkPSJyZWN0MTAzNiIgY2xhc3M9ImNscy0xIiB4PSIxMSIgeT0iMTEiIHdpZHRoPSIzNTgiIGhlaWdodD0iNzkiLz48cGF0aCBpZD0icGF0aDEwMzgiIGNsYXNzPSJjbHMtMiIgZD0iTTgsOFY5M0gzNzJWOFpNMzY5LDkwSDExVjExSDM2OVoiLz48cGF0aCBpZD0icGF0aDEwNDAiIGNsYXNzPSJjbHMtMyIgZD0iTTAsMFYxMDFIMzgwVjBaTTM3Miw5M0g4VjhIMzcyWiIvPjwvZz48L2c+PC9zdmc+\",\"srcOrientation\":\"Right\"},\"position\":[0,0,1,1],\"scaleMode\":\"0\"}},{\"name\":\"ForegroundImageComponent\",\"settings\":{\"angle\":0,\"image\":{\"size\":[0,0],\"src\":\"default\"},\"isForeground\":1,\"position\":[0,0,1,1],\"scaleMode\":\"0\"}}],\"derived\":{\"blockParameters\":{\"fixedAspectRatio\":\"on\",\"format\":\"short\",\"formatString\":\"%d\"}},\"settings\":{\"BindingType\":\"signal\",\"aspectRatio\":1.032258064516129,\"backgroundColor\":[0,0,0,\"1\"],\"backgroundOffset\":0.14,\"backgroundOpacity\":1,\"fixedAspectRatio\":\"on\",\"showBackgroundColor\":false,\"value\":0,\"version\":\"R2023b\"},\"type\":\"Display\"}"
  panelInfo : PanelWebBlock  Tag=HiddenForWebPanel  PanelInfo="{\"compacted\":false,\"height\":451,\"isActiveTab\":true,\"labels\":{\"label1776603344\":{\"deleted\":false,\"left\":526,\"settings\":{\"backgroundColor\":\"rgba(0, 0, 0, 0)\",\"bold\":false,\"font\":\"Arial\",\"fontColor\":\"black\",\"fontSize\":0.9,\"italicized\":false,\"underlined\":false},\"text\":\"Minimum cell voltage (V)\",\"top\":159},\"label2089421704\":{\"deleted\":false,\"left\":638,\"settings\":{\"backgroundColor\":\"rgba(0, 0, 0, 0)\",\"bold\":false,\"font\":\"Arial\",\"fontColor\":\"black\",\"fontSize\":0.9,\"italicized\":false,\"underlined\":false},\"text\":\"Undervoltage\",\"top\":388},\"label2532292209\":{\"deleted\":false,\"left\":360,\"settings\":{\"backgroundColor\":\"rgba(0, 0, 0, 0)\",\"bold\":false,\"font\":\"Arial\",\"fontColor\":\"black\",\"fontSize\":0.9,\"italicized\":false,\"underlined\":false},\"text\":\"Requested current (A)\",\"top\":33},\"label3211207757\":{\"deleted\":false,\"left\":430,\"settings\":{\"backgroundColor\":\"rgba(0, 0, 0, 0)\",\"bold\":false,\"font\":\"Arial\",\"fontColor\":\"black\",\"fontSize\":0.9,\"italicized\":false,\"underlined\":false},\"text\":\" Discharge allowed\",\"top\":284},\"label3844723304\":{\"deleted\":false,\"left\":712,\"settings\":{\"backgroundColor\":\"rgba(0, 0, 0, 0)\",\"bold\":false,\"font\":\"Arial\",\"fontColor\":\"black\",\"fontSize\":0.9,\"italicized\":false,\"underlined\":false},\"text\":\"Pack voltage (V)\",\"top\":162},\"label4628971052\":{\"deleted\":false,\"left\":278,\"settings\":{\"backgroundColor\":\"rgba(0, 0, 0, 0)\",\"bold\":false,\"font\":\"Arial\",\"fontColor\":\"black\",\"fontSize\":0.9,\"italicized\":false,\"underlined\":false},\"text\":\"Temperature (°C)\",\"top\":228},\"label4757796133\":{\"deleted\":false,\"left\":669,\"settings\":{\"backgroundColor\":\"rgba(0, 0, 0, 0)\",\"bold\":false,\"font\":\"Arial\",\"fontColor\":\"black\",\"fontSize\":0.9,\"italicized\":false,\"underlined\":false},\"text\":\"Reset overcurrent\",\"top\":34},\"label4948322395\":{\"deleted\":false,\"left\":763,\"settings\":{\"backgroundColor\":\"rgba(0, 0, 0, 0)\",\"bold\":false,\"font\":\"Arial\",\"fontColor\":\"black\",\"fontSize\":0.9,\"italicized\":false,\"underlined\":false},\"text\":\"Overcurrent\",\"top\":388},\"label4984516083\":{\"deleted\":false,\"left\":307,\"settings\":{\"backgroundColor\":\"rgba(0, 0, 0, 0)\",\"bold\":false,\"font\":\"Arial\",\"fontColor\":\"black\",\"fontSize\":0.9,\"italicized\":false,\"underlined\":false},\"text\":\"Charge allowed\",\"top\":284},\"label5697576641\":{\"deleted\":false,\"left\":216,\"settings\":{\"backgroundColor\":\"rgba(0, 0, 0, 0)\",\"bold\":false,\"font\":\"Arial\",\"fontColor\":\"black\",\"fontSize\":0.9,\"italicized\":false,\"underlined\":false},\"text\":\"Requested current (A)\",\"top\":160},\"label5750223172\":{\"deleted\":false,\"left\":374,\"settings\":{\"backgroundColor\":\"rgba(0, 0, 0, 0)\",\"bold\":false,\"font\":\"Arial\",\"fontColor\":\"black\",\"fontSize\":0.9,\"italicized\":false,\"underlined\":false},\"text\":\"Applied current (A)\",\"top\":161},\"label7054374091\":{\"deleted\":false,\"left\":131,\"settings\":{\"backgroundColor\":\"rgba(0, 0, 0, 0)\",\"bold\":false,\"font\":\"Arial\",\"fontColor\":\"black\",\"fontSize\":0.9,\"italicized\":false,\"underlined\":false},\"text\":\"Temperature (°C)\",\"top\":31},\"label7158709923\":{\"deleted\":false,\"left\":18,\"settings\":{\"backgroundColor\":\"rgba(0, 0, 0, 0)\",\"bold\":false,\"font\":\"Arial\",\"fontColor\":\"black\",\"fontSize\":0.9,\"italicized\":false,\"underlined\":false},\"text\":\"Minimum estimated SOC (%)\",\"top\":160},\"label7430554816\":{\"deleted\":false,\"left\":464,\"settings\":{\"backgroundColor\":\"rgba(0, 0, 0, 0)\",\"bold\":false,\"font\":\"Arial\",\"fontColor\":\"black\",\"fontSize\":0.9,\"italicized\":false,\"underlined\":false},\"text\":\"Maximum cell voltage (V)\",\"top\":226},\"label9043419208\":{\"deleted\":false,\"left\":444,\"settings\":{\"backgroundColor\":\"rgba(0, 0, 0, 0)\",\"bold\":false,\"font\":\"Arial\",\"fontColor\":\"black\",\"fontSize\":0.9,\"italicized\":false,\"underlined\":false},\"text\":\" Discharge temperature fault\",\"top\":386},\"label9244135669\":{\"deleted\":false,\"left\":151,\"settings\":{\"backgroundColor\":\"rgba(0, 0, 0, 0)\",\"bold\":false,\"font\":\"Arial\",\"fontColor\":\"black\",\"fontSize\":0.9,\"italicized\":false,\"underlined\":false},\"text\":\"Charge temperature fault\",\"top\":386},\"label9704342591\":{\"deleted\":false,\"left\":352,\"settings\":{\"backgroundColor\":\"rgba(0, 0, 0, 0)\",\"bold\":false,\"font\":\"Arial\",\"fontColor\":\"black\",\"fontSize\":0.9,\"italicized\":false,\"underlined\":false},\"text\":\"Overvoltage\",\"top\":387}},\"left\":75,\"name\":\"Panel\",\"panelId\":\"panelId-01a7e0ec-c42e-414d-a098-7f8dff93f820\",\"tabIndex\":0,\"tabbedSetId\":\"tabbedSet5448519163\",\"top\":79,\"type\":\"panel\",\"version\":\"2019b\",\"visible\":true,\"width\":860,\"zIndex\":1500002}"  PanelSnapshot=<binary blob, 169476 chars, not shown>
  request : ToggleSwitchBlock  Tag=HiddenForWebPanel  PanelInfo="{\"height\":75,\"left\":647,\"panelId\":\"panelId-01a7e0ec-c42e-414d-a098-7f8dff93f820\",\"top\":58,\"type\":\"panelChild\",\"version\":\"2019b\",\"width\":155,\"zIndex\":1500018}"
